simulink model "GRID_SUPPORTED_WIND_R1"  (R2026a)
settings: Solver=ode14x  StopTime=1.1  FixedStep=1e-5
InitFcn:
  | setup_v2_paths; init_grid_supported_integration;
undefined symbols (not defined in the file): Base, Control, Converter, Drive, Filter, PMSG, V2, Wind
libraries: nesl_utility x21, ee_lib x14, fl_lib x6, simulink x1
(part 2 of 2)

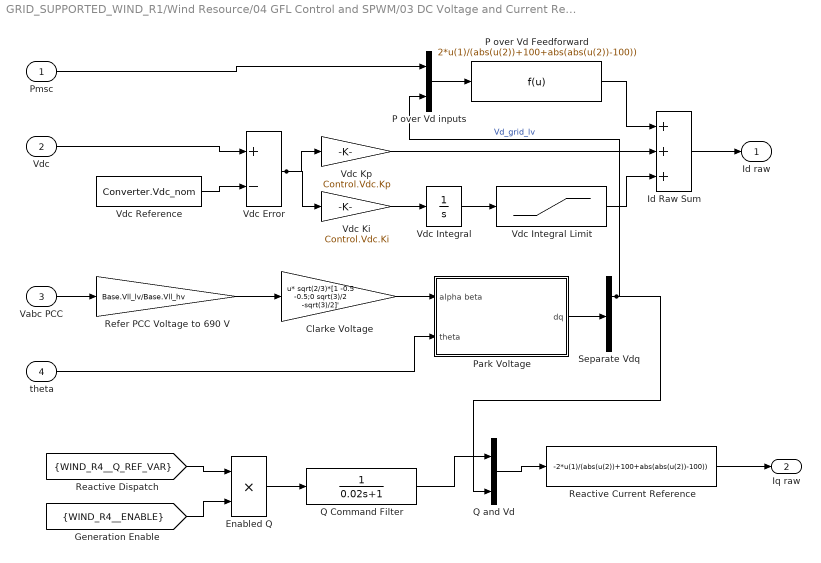
== system GRID_SUPPORTED_WIND_R1/Wind Resource/04 GFL Control and SPWM/03 DC Voltage and Current Reference ==
  Pmsc : Inport
  Vdc : Inport  Port=2
  Vabc PCC : Inport  Port=3
  theta : Inport  Port=4
  Clarke Voltage : Gain  Gain=sqrt(2/3)*[1 -0.5 -0.5;0 sqrt(3)/2 -sqrt(3)/2]'  Multiplication=Matrix(u*K)
  Enabled Q : Product
  Id Raw Sum : Sum  Inputs=+++
  P over Vd Feedforward : Fcn  Expr=2*u(1)/(abs(u(2))+100+abs(abs(u(2))-100))
  P over Vd inputs : Mux  Inputs=2
  Park Voltage : Subsystem
  Q Command Filter : TransferFcn  Numerator=1  Denominator=[0.02 1]
  Q and Vd : Mux  Inputs=2
  Reactive Current Reference : Fcn  Expr=-2*u(1)/(abs(u(2))+100+abs(abs(u(2))-100))
  Refer PCC Voltage to 690 V : Gain  Gain=Base.Vll_lv/Base.Vll_hv
  Separate Vdq : Demux  Outputs=2
  Vdc Error : Sum  Inputs=+-
  Vdc Integral : Integrator
  Vdc Integral Limit : Saturate  UpperLimit=Control.Vdc.IntegratorLimit  LowerLimit=-Control.Vdc.IntegratorLimit
  Vdc Ki : Gain  Gain=Control.Vdc.Ki
  Vdc Kp : Gain  Gain=Control.Vdc.Kp
  Vdc Reference : Constant  Value=Converter.Vdc_nom
  Id raw : Outport
  Iq raw : Outport  Port=2
  wires:
  Id Raw Sum/1 -> Id raw/1
  Vdc Integral Limit/1 -> Id Raw Sum/3
  Vdc Kp/1 -> Id Raw Sum/2
  P over Vd Feedforward/1 -> Id Raw Sum/1
  Vdc Integral/1 -> Vdc Integral Limit/1
  Vdc Ki/1 -> Vdc Integral/1
  Vdc Error/1 -> Vdc Ki/1, Vdc Kp/1
  Vdc Reference/1 -> Vdc Error/2
  Vdc/1 -> Vdc Error/1
  P over Vd inputs/1 -> P over Vd Feedforward/1
  Separate Vdq/1 -> P over Vd inputs/2, Q and Vd/2  "Vd_grid_lv"
  Pmsc/1 -> P over Vd inputs/1
  Park Voltage/1(dq) -> Separate Vdq/1
  theta/1 -> Park Voltage/2(theta)
  Clarke Voltage/1 -> Park Voltage/1(alpha beta)
  Refer PCC Voltage to 690 V/1 -> Clarke Voltage/1
  Vabc PCC/1 -> Refer PCC Voltage to 690 V/1
  [WIND_R4__Q_REF_VAR] -> Enabled Q/1
  [WIND_R4__ENABLE] -> Enabled Q/2
  Enabled Q/1 -> Q Command Filter/1
  Q Command Filter/1 -> Q and Vd/1
  Q and Vd/1 -> Reactive Current Reference/1
  Reactive Current Reference/1 -> Iq raw/1

== system GRID_SUPPORTED_WIND_R1/Wind Resource/04 GFL Control and SPWM/04 Circular Current Limiter ==
  note: Circular physical limit preserves dq direction: [Id,Iq]_lim=min(1,Imax/|I*|)[Id,Iq].
  Id raw : Inport
  Iq raw : Inport  Port=2
  Id squared : Product
  Iq squared : Product
  Limit Id : Product
  Limit Iq : Product
  Limiter Active : simulink/Logic and Bit Operations/Compare To Constant  relop=<  const=0.999999  OutDataTypeStr=boolean
  Magnitude : Sqrt
  Magnitude squared : Sum
  Scale factor : Fcn  Expr=0.5*(1+2*Converter.IdqMax/(u+1e-6+abs(u-1e-6))-abs(1-2*Converter.IdqMax/(u+1e-6+abs(u-1e-6))))
  Id limited : Outport
  Iq limited : Outport  Port=2
  Limit active : Outport  Port=3
  tag scope: WIND_R4__ID_REF_RESOURCE=scoped, WIND_R4__IQ_REF_RESOURCE=scoped
  wires:
  Limiter Active/1 -> Limit active/1
  Limit Iq/1 -> Iq limited/1
  Limit Id/1 -> Id limited/1
  [WIND_R4__IQ_RAW_LOCAL] -> Limit Iq/2
  Scale factor/1 -> Limiter Active/1, Limit Iq/1, Limit Id/2
  [WIND_R4__ID_RAW_LOCAL] -> Limit Id/1
  Magnitude/1 -> Scale factor/1  "CurrentUtilization"
  Magnitude squared/1 -> Magnitude/1
  Iq squared/1 -> Magnitude squared/2
  Id squared/1 -> Magnitude squared/1
  Iq raw/1 -> [WIND_R4__IQ_RAW_LOCAL], Iq squared/2, Iq squared/1, [WIND_R4__IQ_REF_RESOURCE]
  Id raw/1 -> [WIND_R4__ID_RAW_LOCAL], Id squared/2, Id squared/1, [WIND_R4__ID_REF_RESOURCE]

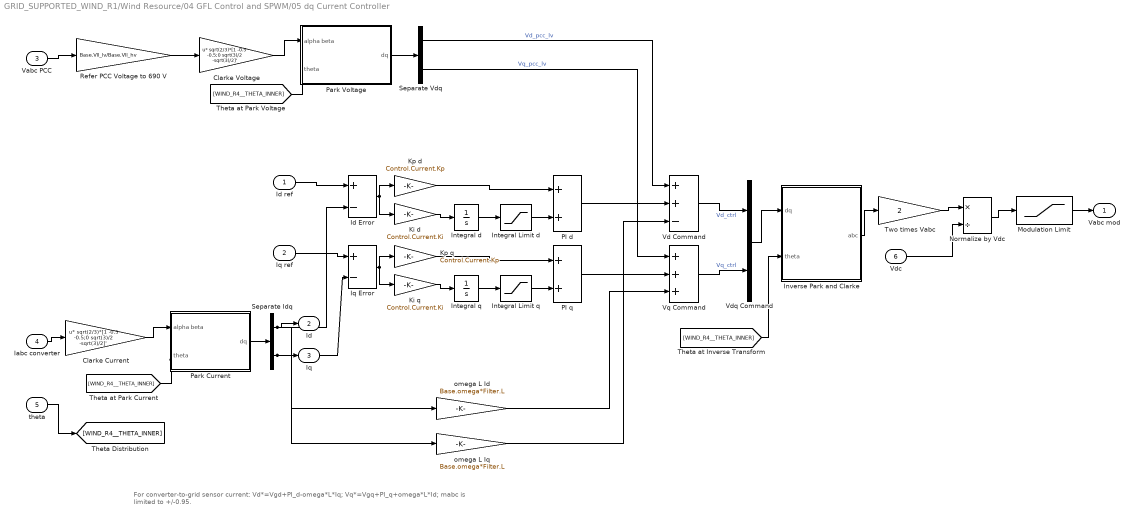
== system GRID_SUPPORTED_WIND_R1/Wind Resource/04 GFL Control and SPWM/05 dq Current Controller ==
  note: For converter-to-grid sensor current: Vd*=Vgd+PI_d-omega*L*Iq; Vq*=Vgq+PI_q+omega*L*Id; mabc is limited to +/-0.95.
  Id ref : Inport
  Iq ref : Inport  Port=2
  Vabc PCC : Inport  Port=3
  Iabc converter : Inport  Port=4
  theta : Inport  Port=5
  Vdc : Inport  Port=6
  Clarke Current : Gain  Gain=sqrt(2/3)*[1 -0.5 -0.5;0 sqrt(3)/2 -sqrt(3)/2]'  Multiplication=Matrix(u*K)
  Clarke Voltage : Gain  Gain=sqrt(2/3)*[1 -0.5 -0.5;0 sqrt(3)/2 -sqrt(3)/2]'  Multiplication=Matrix(u*K)
  Id Error : Sum  Inputs=+-
  Integral Limit d : Saturate  UpperLimit=Control.Current.IntegratorLimitV  LowerLimit=-Control.Current.IntegratorLimitV
  Integral Limit q : Saturate  UpperLimit=Control.Current.IntegratorLimitV  LowerLimit=-Control.Current.IntegratorLimitV
  Integral d : Integrator
  Integral q : Integrator
  Inverse Park and Clarke : Subsystem
  Iq Error : Sum  Inputs=+-
  Ki d : Gain  Gain=Control.Current.Ki
  Ki q : Gain  Gain=Control.Current.Ki
  Kp d : Gain  Gain=Control.Current.Kp
  Kp q : Gain  Gain=Control.Current.Kp
  Modulation Limit : Saturate  UpperLimit=Converter.ModulationMax  LowerLimit=-Converter.ModulationMax
  Normalize by Vdc : Product  Inputs=*/
  PI d : Sum
  PI q : Sum
  Park Current : Subsystem
  Park Voltage : Subsystem
  Refer PCC Voltage to 690 V : Gain  Gain=Base.Vll_lv/Base.Vll_hv
  Separate Idq : Demux  Outputs=2
  Separate Vdq : Demux  Outputs=2
  Two times Vabc : Gain  Gain=2
  Vd Command : Sum  Inputs=++-
  Vdq Command : Mux  Inputs=2
  Vq Command : Sum  Inputs=+++
  omega L Id : Gain  Gain=Base.omega*Filter.L
  omega L Iq : Gain  Gain=Base.omega*Filter.L
  Vabc mod : Outport
  Id : Outport  Port=2
  Iq : Outport  Port=3
  wires:
  Modulation Limit/1 -> Vabc mod/1
  Normalize by Vdc/1 -> Modulation Limit/1
  Vdc/1 -> Normalize by Vdc/2
  Two times Vabc/1 -> Normalize by Vdc/1
  Inverse Park and Clarke/1(abc) -> Two times Vabc/1
  theta/1 -> [WIND_R4__THETA_INNER]
  [WIND_R4__THETA_INNER] -> Inverse Park and Clarke/2(theta)
  Vdq Command/1 -> Inverse Park and Clarke/1(dq)
  Vq Command/1 -> Vdq Command/2  "Vq_ctrl"
  Vd Command/1 -> Vdq Command/1  "Vd_ctrl"
  omega L Id/1 -> Vq Command/3
  PI q/1 -> Vq Command/2
  Separate Vdq/2 -> Vq Command/1  "Vq_pcc_lv"
  omega L Iq/1 -> Vd Command/3
  PI d/1 -> Vd Command/2
  Separate Vdq/1 -> Vd Command/1  "Vd_pcc_lv"
  Integral Limit q/1 -> PI q/2
  Integral q/1 -> Integral Limit q/1
  Kp q/1 -> PI q/1
  Ki q/1 -> Integral q/1
  Iq Error/1 -> Ki q/1, Kp q/1
  Integral Limit d/1 -> PI d/2
  Integral d/1 -> Integral Limit d/1
  Kp d/1 -> PI d/1
  Ki d/1 -> Integral d/1
  Id Error/1 -> Ki d/1, Kp d/1
  Separate Idq/2 -> Iq/1, omega L Iq/1, Iq Error/2
  Iq ref/1 -> Iq Error/1
  Separate Idq/1 -> Id/1, omega L Id/1, Id Error/2
  Id ref/1 -> Id Error/1
  Park Current/1(dq) -> Separate Idq/1
  [WIND_R4__THETA_INNER] -> Park Current/2(theta)
  Clarke Current/1 -> Park Current/1(alpha beta)
  Iabc converter/1 -> Clarke Current/1
  Park Voltage/1(dq) -> Separate Vdq/1
  [WIND_R4__THETA_INNER] -> Park Voltage/2(theta)
  Clarke Voltage/1 -> Park Voltage/1(alpha beta)
  Refer PCC Voltage to 690 V/1 -> Clarke Voltage/1
  Vabc PCC/1 -> Refer PCC Voltage to 690 V/1

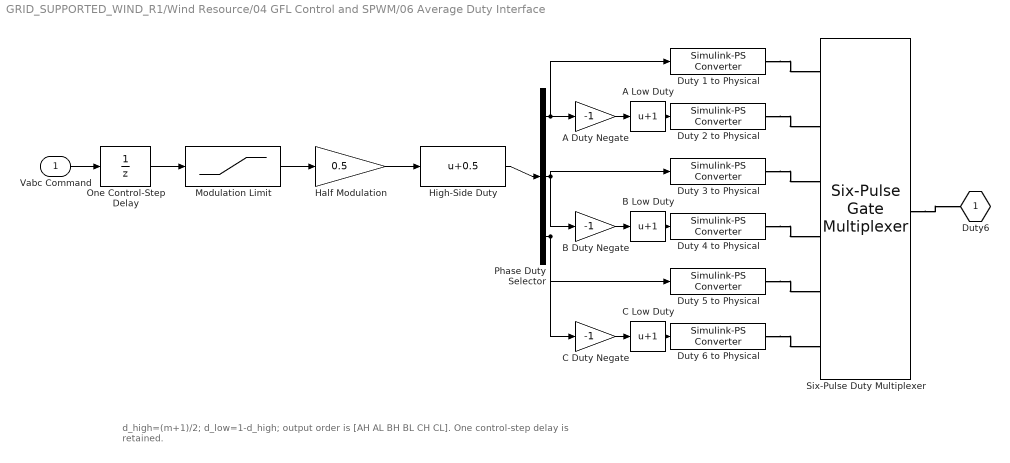
== system GRID_SUPPORTED_WIND_R1/Wind Resource/04 GFL Control and SPWM/06 Average Duty Interface ==
  note: d_high=(m+1)/2; d_low=1-d_high; output order is [AH AL BH BL CH CL]. One control-step delay is retained.
  Vabc Command : Inport
  A Duty Negate : Gain  Gain=-1
  A Low Duty : Bias  Bias=1  SaturateOnIntegerOverflow=off
  B Duty Negate : Gain  Gain=-1
  B Low Duty : Bias  Bias=1  SaturateOnIntegerOverflow=off
  C Duty Negate : Gain  Gain=-1
  C Low Duty : Bias  Bias=1  SaturateOnIntegerOverflow=off
  Duty 1 to Physical : nesl_utility/Simulink-PS Converter  PhysicalDomain=network_engine_domain  SubClassName=ps_input  LeftPortType=input  RightPortType=output  PseudoPeriodic=off  Frequencies=[]  NoiseDistribution=none  NoiseParameters=[]  Unit=V  AffineConversion=off  FilteringAndDerivatives=provide  SimscapeFilterOrder=1  InputFilterTimeConstant=0.001  UdotUserProvided=0
  Duty 2 to Physical : nesl_utility/Simulink-PS Converter  PhysicalDomain=network_engine_domain  SubClassName=ps_input  LeftPortType=input  RightPortType=output  PseudoPeriodic=off  Frequencies=[]  NoiseDistribution=none  NoiseParameters=[]  Unit=V  AffineConversion=off  FilteringAndDerivatives=provide  SimscapeFilterOrder=1  InputFilterTimeConstant=0.001  UdotUserProvided=0
  Duty 3 to Physical : nesl_utility/Simulink-PS Converter  PhysicalDomain=network_engine_domain  SubClassName=ps_input  LeftPortType=input  RightPortType=output  PseudoPeriodic=off  Frequencies=[]  NoiseDistribution=none  NoiseParameters=[]  Unit=V  AffineConversion=off  FilteringAndDerivatives=provide  SimscapeFilterOrder=1  InputFilterTimeConstant=0.001  UdotUserProvided=0
  Duty 4 to Physical : nesl_utility/Simulink-PS Converter  PhysicalDomain=network_engine_domain  SubClassName=ps_input  LeftPortType=input  RightPortType=output  PseudoPeriodic=off  Frequencies=[]  NoiseDistribution=none  NoiseParameters=[]  Unit=V  AffineConversion=off  FilteringAndDerivatives=provide  SimscapeFilterOrder=1  InputFilterTimeConstant=0.001  UdotUserProvided=0
  Duty 5 to Physical : nesl_utility/Simulink-PS Converter  PhysicalDomain=network_engine_domain  SubClassName=ps_input  LeftPortType=input  RightPortType=output  PseudoPeriodic=off  Frequencies=[]  NoiseDistribution=none  NoiseParameters=[]  Unit=V  AffineConversion=off  FilteringAndDerivatives=provide  SimscapeFilterOrder=1  InputFilterTimeConstant=0.001  UdotUserProvided=0
  Duty 6 to Physical : nesl_utility/Simulink-PS Converter  PhysicalDomain=network_engine_domain  SubClassName=ps_input  LeftPortType=input  RightPortType=output  PseudoPeriodic=off  Frequencies=[]  NoiseDistribution=none  NoiseParameters=[]  Unit=V  AffineConversion=off  FilteringAndDerivatives=provide  SimscapeFilterOrder=1  InputFilterTimeConstant=0.001  UdotUserProvided=0
  Half Modulation : Gain  Gain=0.5
  High-Side Duty : Bias  Bias=0.5  SaturateOnIntegerOverflow=off
  Modulation Limit : Saturate  UpperLimit=Converter.ModulationMax  LowerLimit=-Converter.ModulationMax
  One Control-Step Delay : UnitDelay  InitialCondition=[0 0 0]  SampleTime=Control.Ts
  Phase Duty Selector : Demux  Outputs=3
  Six-Pulse Duty Multiplexer : ee_lib/Semiconductors & Converters/Converters/Six-Pulse Gate Multiplexer  port_option=ee.enum.controlport.ps
  Duty6 : PMIOPort  Side=Right
  wires:
  C Low Duty/1 -> Duty 6 to Physical/1
  C Duty Negate/1 -> C Low Duty/1
  Phase Duty Selector/3 -> C Duty Negate/1, Duty 5 to Physical/1
  B Low Duty/1 -> Duty 4 to Physical/1
  B Duty Negate/1 -> B Low Duty/1
  Phase Duty Selector/2 -> B Duty Negate/1, Duty 3 to Physical/1
  A Low Duty/1 -> Duty 2 to Physical/1
  A Duty Negate/1 -> A Low Duty/1
  Phase Duty Selector/1 -> A Duty Negate/1, Duty 1 to Physical/1
  High-Side Duty/1 -> Phase Duty Selector/1
  Half Modulation/1 -> High-Side Duty/1
  Modulation Limit/1 -> Half Modulation/1
  One Control-Step Delay/1 -> Modulation Limit/1
  Vabc Command/1 -> One Control-Step Delay/1
  connections:
  Six-Pulse Duty Multiplexer/RConn1 -- Duty6/RConn1
  Duty 6 to Physical/RConn1 -- Six-Pulse Duty Multiplexer/LConn6
  Duty 5 to Physical/RConn1 -- Six-Pulse Duty Multiplexer/LConn5
  Duty 4 to Physical/RConn1 -- Six-Pulse Duty Multiplexer/LConn4
  Duty 3 to Physical/RConn1 -- Six-Pulse Duty Multiplexer/LConn3
  Duty 2 to Physical/RConn1 -- Six-Pulse Duty Multiplexer/LConn2
  Duty 1 to Physical/RConn1 -- Six-Pulse Duty Multiplexer/LConn1

== system GRID_SUPPORTED_WIND_R1/Wind Resource/Resource Status/MSC Available Power ==
  In1 : Inport
  Available Airgap Power : Product
  Available Auxiliary Loss : Bias  Bias=-PMSG.loss_constant_W  SaturateOnIntegerOverflow=off
  Available MPPT Torque : Fcn  Expr=0.5*(Wind.Kopt_Nm_per_rad_s2*u^2+PMSG.torque_limit_Nm-abs(Wind.Kopt_Nm_per_rad_s2*u^2-PMSG.torque_limit_Nm))
  Available MSC Efficiency : Gain  Gain=PMSG.msc_efficiency
  Available Machine Power : Sum  Inputs=+-
  Available Power Limit : Saturate  UpperLimit=PMSG.Sn_W  LowerLimit=0
  Available iq : Gain  Gain=-1/(1.5*PMSG.pole_pairs*PMSG.psi_f_Wb)
  Available iq squared : Product
  Estimated Copper Loss : Gain  Gain=1.5*PMSG.Rs_ohm
  available_power_W : Outport
  wires:
  Available Machine Power/1 -> Available MSC Efficiency/1
  Estimated Copper Loss/1 -> Available Machine Power/2
  Available iq squared/1 -> Estimated Copper Loss/1
  Available Airgap Power/1 -> Available Machine Power/1
  Available Power Limit/1 -> available_power_W/1  "available_power_W"
  Available MSC Efficiency/1 -> Available Auxiliary Loss/1
  Available MPPT Torque/1 -> Available iq/1, Available Airgap Power/1
  Available Auxiliary Loss/1 -> Available Power Limit/1
  Available iq/1 -> Available iq squared/2, Available iq squared/1
  In1/1 -> Available MPPT Torque/1, Available Airgap Power/2

== system GRID_SUPPORTED_WIND_R1/Wind Resource/02 PMSG dq Machine and Average MSC/01 Torque and Current References/Dispatch Torque Limit ==
  In1 : Inport
  In2 : Inport  Port=2
  Dispatch Inputs : Mux
  Dispatch Torque Cap : Fcn  Expr=0.5*(u(1)+u(2)/u(3)-abs(u(1)-u(2)/u(3)))*u(4)
  Speed Floor : Saturate  UpperLimit=inf  LowerLimit=PMSG.speed_floor_rad_s
  Out1 : Outport
  wires:
  Dispatch Torque Cap/1 -> Out1/1
  Dispatch Inputs/1 -> Dispatch Torque Cap/1
  In2/1 -> Dispatch Inputs/1
  [WIND_R4__ENABLE] -> Dispatch Inputs/4
  Speed Floor/1 -> Dispatch Inputs/3
  [WIND_R4__DISPATCH_W] -> Dispatch Inputs/2
  In1/1 -> Speed Floor/1

== system GRID_SUPPORTED_WIND_R1/Wind Resource/03 DC Link and Two-Level GSC/Converter AC Measurement/Line Voltage Calculation ==
  Vabc : Inport
  Separate abc : Demux  Outputs=3
  Vab = Va - Vb : Sum  Inputs=+-
  Vab Vbc Vca : Mux  Inputs=3
  Vbc = Vb - Vc : Sum  Inputs=+-
  Vca = Vc - Va : Sum  Inputs=+-
  Vll : Outport
  wires:
  Vab Vbc Vca/1 -> Vll/1  "Vll_inv"
  Vca = Vc - Va/1 -> Vab Vbc Vca/3
  Vbc = Vb - Vc/1 -> Vab Vbc Vca/2
  Vab = Va - Vb/1 -> Vab Vbc Vca/1
  Separate abc/3 -> Vca = Vc - Va/1, Vbc = Vb - Vc/2
  Separate abc/2 -> Vbc = Vb - Vc/1, Vab = Va - Vb/2
  Separate abc/1 -> Vca = Vc - Va/2, Vab = Va - Vb/1
  Vabc/1 -> Separate abc/1

== system GRID_SUPPORTED_WIND_R1/Wind Resource/04 GFL Control and SPWM/01 Measurements and dq/Current alpha beta to dq ==
  alpha beta : Inport
  theta : Inport  Port=2
  Separate alpha beta : Demux  Outputs=2
  alpha cos : Product
  alpha sin : Product
  beta cos : Product
  beta sin : Product
  cos theta : Trigonometry  Operator=cos
  d = alpha cos + beta sin : Sum
  dq vector : Mux  Inputs=2
  q = -alpha sin + beta cos : Sum  Inputs=-+
  sin theta : Trigonometry
  dq : Outport
  wires:
  dq vector/1 -> dq/1
  q = -alpha sin + beta cos/1 -> dq vector/2
  d = alpha cos + beta sin/1 -> dq vector/1
  beta cos/1 -> q = -alpha sin + beta cos/2
  alpha sin/1 -> q = -alpha sin + beta cos/1
  beta sin/1 -> d = alpha cos + beta sin/2
  alpha cos/1 -> d = alpha cos + beta sin/1
  sin theta/1 -> alpha sin/2, beta sin/2
  Separate alpha beta/2 -> beta cos/1, beta sin/1
  cos theta/1 -> beta cos/2, alpha cos/2
  Separate alpha beta/1 -> alpha sin/1, alpha cos/1
  theta/1 -> sin theta/1, cos theta/1
  alpha beta/1 -> Separate alpha beta/1

== system GRID_SUPPORTED_WIND_R1/Wind Resource/04 GFL Control and SPWM/01 Measurements and dq/Voltage alpha beta to dq ==
  alpha beta : Inport
  theta : Inport  Port=2
  Separate alpha beta : Demux  Outputs=2
  alpha cos : Product
  alpha sin : Product
  beta cos : Product
  beta sin : Product
  cos theta : Trigonometry  Operator=cos
  d = alpha cos + beta sin : Sum
  dq vector : Mux  Inputs=2
  q = -alpha sin + beta cos : Sum  Inputs=-+
  sin theta : Trigonometry
  dq : Outport
  wires:
  dq vector/1 -> dq/1
  q = -alpha sin + beta cos/1 -> dq vector/2
  d = alpha cos + beta sin/1 -> dq vector/1
  beta cos/1 -> q = -alpha sin + beta cos/2
  alpha sin/1 -> q = -alpha sin + beta cos/1
  beta sin/1 -> d = alpha cos + beta sin/2
  alpha cos/1 -> d = alpha cos + beta sin/1
  sin theta/1 -> alpha sin/2, beta sin/2
  Separate alpha beta/2 -> beta cos/1, beta sin/1
  cos theta/1 -> beta cos/2, alpha cos/2
  Separate alpha beta/1 -> alpha sin/1, alpha cos/1
  theta/1 -> sin theta/1, cos theta/1
  alpha beta/1 -> Separate alpha beta/1

== system GRID_SUPPORTED_WIND_R1/Wind Resource/04 GFL Control and SPWM/02 Synchronization SRF-PLL/PCC Voltage Prefilter ==
  abc raw : Inport
  Filtered abc : Mux  Inputs=3
  Phase A LPF : TransferFcn  Numerator=[2*pi*Control.PLL.VoltagePrefilterHz]  Denominator=[1 2*pi*Control.PLL.VoltagePrefilterHz]
  Phase B LPF : TransferFcn  Numerator=[2*pi*Control.PLL.VoltagePrefilterHz]  Denominator=[1 2*pi*Control.PLL.VoltagePrefilterHz]
  Phase C LPF : TransferFcn  Numerator=[2*pi*Control.PLL.VoltagePrefilterHz]  Denominator=[1 2*pi*Control.PLL.VoltagePrefilterHz]
  Separate abc : Demux  Outputs=3
  abc filtered : Outport
  wires:
  Filtered abc/1 -> abc filtered/1
  abc raw/1 -> Separate abc/1
  Phase C LPF/1 -> Filtered abc/3
  Separate abc/3 -> Phase C LPF/1
  Phase B LPF/1 -> Filtered abc/2
  Separate abc/2 -> Phase B LPF/1
  Phase A LPF/1 -> Filtered abc/1
  Separate abc/1 -> Phase A LPF/1

== system GRID_SUPPORTED_WIND_R1/Wind Resource/04 GFL Control and SPWM/02 Synchronization SRF-PLL/Park Voltage ==
  alpha beta : Inport
  theta : Inport  Port=2
  Separate alpha beta : Demux  Outputs=2
  alpha cos : Product
  alpha sin : Product
  beta cos : Product
  beta sin : Product
  cos theta : Trigonometry  Operator=cos
  d = alpha cos + beta sin : Sum
  dq vector : Mux  Inputs=2
  q = -alpha sin + beta cos : Sum  Inputs=-+
  sin theta : Trigonometry
  dq : Outport
  wires:
  dq vector/1 -> dq/1
  q = -alpha sin + beta cos/1 -> dq vector/2
  d = alpha cos + beta sin/1 -> dq vector/1
  beta cos/1 -> q = -alpha sin + beta cos/2
  alpha sin/1 -> q = -alpha sin + beta cos/1
  beta sin/1 -> d = alpha cos + beta sin/2
  alpha cos/1 -> d = alpha cos + beta sin/1
  sin theta/1 -> alpha sin/2, beta sin/2
  Separate alpha beta/2 -> beta cos/1, beta sin/1
  cos theta/1 -> beta cos/2, alpha cos/2
  Separate alpha beta/1 -> alpha sin/1, alpha cos/1
  theta/1 -> sin theta/1, cos theta/1
  alpha beta/1 -> Separate alpha beta/1

== system GRID_SUPPORTED_WIND_R1/Wind Resource/04 GFL Control and SPWM/03 DC Voltage and Current Reference/Park Voltage ==
  alpha beta : Inport
  theta : Inport  Port=2
  Separate alpha beta : Demux  Outputs=2
  alpha cos : Product
  alpha sin : Product
  beta cos : Product
  beta sin : Product
  cos theta : Trigonometry  Operator=cos
  d : Sum
  dq vector : Mux  Inputs=2
  q : Sum  Inputs=-+
  sin theta : Trigonometry
  dq : Outport
  wires:
  dq vector/1 -> dq/1
  q/1 -> dq vector/2
  d/1 -> dq vector/1
  beta cos/1 -> q/2
  alpha sin/1 -> q/1
  beta sin/1 -> d/2
  alpha cos/1 -> d/1
  sin theta/1 -> alpha sin/2, beta sin/2
  Separate alpha beta/2 -> beta cos/1, beta sin/1
  cos theta/1 -> beta cos/2, alpha cos/2
  Separate alpha beta/1 -> alpha sin/1, alpha cos/1
  theta/1 -> sin theta/1, cos theta/1
  alpha beta/1 -> Separate alpha beta/1

== system GRID_SUPPORTED_WIND_R1/Wind Resource/04 GFL Control and SPWM/05 dq Current Controller/Inverse Park and Clarke ==
  dq : Inport
  theta : Inport  Port=2
  Inverse Clarke : Gain  Gain=sqrt(2/3)*[1 -0.5 -0.5;0 sqrt(3)/2 -sqrt(3)/2]  Multiplication=Matrix(u*K)
  Separate dq : Demux  Outputs=2
  alpha : Sum  Inputs=+-
  alpha beta : Mux  Inputs=2
  beta : Sum
  cos theta : Trigonometry  Operator=cos
  d cos : Product
  d sin : Product
  q cos : Product
  q sin : Product
  sin theta : Trigonometry
  abc : Outport
  wires:
  Inverse Clarke/1 -> abc/1
  alpha beta/1 -> Inverse Clarke/1
  beta/1 -> alpha beta/2
  alpha/1 -> alpha beta/1
  q cos/1 -> beta/2
  d sin/1 -> beta/1
  q sin/1 -> alpha/2
  d cos/1 -> alpha/1
  sin theta/1 -> d sin/2, q sin/2
  Separate dq/2 -> q cos/1, q sin/1
  cos theta/1 -> q cos/2, d cos/2
  Separate dq/1 -> d sin/1, d cos/1
  theta/1 -> sin theta/1, cos theta/1
  dq/1 -> Separate dq/1

== system GRID_SUPPORTED_WIND_R1/Wind Resource/04 GFL Control and SPWM/05 dq Current Controller/Park Current ==
  alpha beta : Inport
  theta : Inport  Port=2
  Separate alpha beta : Demux  Outputs=2
  alpha cos : Product
  alpha sin : Product
  beta cos : Product
  beta sin : Product
  cos theta : Trigonometry  Operator=cos
  d : Sum
  dq vector : Mux  Inputs=2
  q : Sum  Inputs=-+
  sin theta : Trigonometry
  dq : Outport
  wires:
  dq vector/1 -> dq/1
  q/1 -> dq vector/2
  d/1 -> dq vector/1
  beta cos/1 -> q/2
  alpha sin/1 -> q/1
  beta sin/1 -> d/2
  alpha cos/1 -> d/1
  sin theta/1 -> alpha sin/2, beta sin/2
  Separate alpha beta/2 -> beta cos/1, beta sin/1
  cos theta/1 -> beta cos/2, alpha cos/2
  Separate alpha beta/1 -> alpha sin/1, alpha cos/1
  theta/1 -> sin theta/1, cos theta/1
  alpha beta/1 -> Separate alpha beta/1

== system GRID_SUPPORTED_WIND_R1/Wind Resource/04 GFL Control and SPWM/05 dq Current Controller/Park Voltage ==
  alpha beta : Inport
  theta : Inport  Port=2
  Separate alpha beta : Demux  Outputs=2
  alpha cos : Product
  alpha sin : Product
  beta cos : Product
  beta sin : Product
  cos theta : Trigonometry  Operator=cos
  d : Sum
  dq vector : Mux  Inputs=2
  q : Sum  Inputs=-+
  sin theta : Trigonometry
  dq : Outport
  wires:
  dq vector/1 -> dq/1
  q/1 -> dq vector/2
  d/1 -> dq vector/1
  beta cos/1 -> q/2
  alpha sin/1 -> q/1
  beta sin/1 -> d/2
  alpha cos/1 -> d/1
  sin theta/1 -> alpha sin/2, beta sin/2
  Separate alpha beta/2 -> beta cos/1, beta sin/1
  cos theta/1 -> beta cos/2, alpha cos/2
  Separate alpha beta/1 -> alpha sin/1, alpha cos/1
  theta/1 -> sin theta/1, cos theta/1
  alpha beta/1 -> Separate alpha beta/1
